simulink model "FDI_FTC_MKGMPH017"  (R2026a)
settings: Solver=ode4  StopTime=20  FixedStep=sim_dt
PreLoadFcn:
  | %% Quadrotor model parameters
  | % Initialize all model, fault detection, wind and noise settings.
  | 
  | m   = (75 + 45.7)/1000;  % kg
  | l   = 54.33e-3;  % m
  | Jxx = 54737.66e-9;  % kg m^2
  | Jyy = 53435.96e-9;  % kg m^2
  | Jzz = 98934.3e-9;  % kg m^2
  | g   = 9.81;  % m/s^2
  | 
  | %% Motor
  | 
  | kf  = 5e-8;  % N/(rad/s)^2
  | kt  = 0.025*kf;  % N m/(rad/s)^2
  | tau = 0.02;  % s
  | w_max = 2.5*sqrt(m*g/(4*kf));  % rad/s
  | 
  | %% Controller Gains
  | % Attitude controller gains
  | Kp_r = 60*Jxx;   Kd_r = 12*Jxx;  % roll
  | Kp_p = 60*Jyy;   Kd_p = 12*Jyy;  % pitch
  | Kp_y = 3*Jzz;    Kd_y = 2.5*Jzz;  % yaw
  | % Position controller gains
  | Kp_pos  = 1.2;  % [1/s^2]
  | Kd_pos  = 1.8;  % [1/s]
  | a_max   = 2.0;  % acceleration limit
  | att_lim = 25*pi/180;  % roll/pitch limit
  | 
  | %% Initial Conditions
  | p0  = [0; 0; 0];  % m        initial position [x; y; z]
  | v0  = [0; 0; 0];  % m/s      initial velocity
  | q0  = [1; 0; 0; 0];  % initial quaternion
  | om0 = [0; 0; 0];  % rad/s    initial body rates [p; q; r]
  | 
  | %% Test Scenario
  | sim_stop_time = 12;  % s
  | sim_dt        = 0.001;  % s
  | 
  | % Reference step times and values
  | x_step_time   = 3.0;   x_step_value = 10;  % m
  | y_step_time   = 5.0;   y_step_value = 10;  % m
  | z_step_time   = 0.5;   z_step_value = 10;  % m
  | psi_step_time = 7.0;   psi_step_deg = 30;  % degrees
  | psi_step_value = deg2rad(psi_step_deg);  % rad
  | 
  | %% Summary
  | w_hover = sqrt(m*g/(4*kf));
  | fprintf('quad_params: m =  % .4f kg, l = %.4f m, hover speed = %.0f rad/s (limit %.0f rad/s)\n', ...
  |         m, l, w_hover, w_max);
  | if w_hover >= w_max
  |     warning('quad_params: hover speed is above the rotor speed limit - the quad cannot hover.');
  | end
  | 
  | L1_eul = [6; 6; 6];
  | L1_om  = [12; 12; 8];
  | L1_p   = [3; 3; 3];
  | L1_v   = [4; 4; 4];
  | % Observer 2 gains
  | L2_eul = L1_eul;
  | L2_om  = L1_om;
  | L2_p   = L1_p;
  | L2_v   = L1_v;
  | rho_alpha = 0.5;
  | % Residual threshold gains
  | Ku1 = [1; 1; 1; 1; 1];
  | Ku2 = [0.05; 0.05; 0.05; 0.05; 0.05];
  | Ku3 = [0.0004; 0.0004; 0.002; 0.002; 0.002];
  | Kl1 = Ku1;
  | Kl2 = Ku2;
  | Kl3 = Ku3;
  | T_res = 0.015;
  | % Detection thresholds
  | T_flag1     = 0.01;
  | thresh_flag1 = 0.5;
  | T_flag2     = 0.1;
  | thresh_flag2 = 0.7;
  | % Confirmation time
  | t_confirm = 0.5;
  | 
  | %% Wind
  | % Wind controls
  | if ~exist('wind_seed','var'), wind_seed = 1; end
  | wind_on      = 1;
  | wind_t_start = 10;
  | wind_t_end   = 14;
  | rng(wind_seed);
  | % Gust settings
  | wind_n      = 30;
  | wind_Om_rng = [0.1 1.5];
  | wind_alt    = 10;
  | wind_W20    = 10;
  | wind_v0     = [0; 0; 0];
  | % Wind length scales and intensity
  | wind_k    = 0.177 + 0.000823*(wind_alt*3.28084);
  | wind_Lv   = wind_alt;
  | wind_Lh   = wind_Lv/wind_k^1.2;
  | wind_sigv = 0.1*wind_W20;
  | wind_sigh = wind_sigv/wind_k^0.4;
  | % Gust frequency and amplitude
  | wind_Om  = sort(wind_Om_rng(1) + diff(wind_Om_rng)*rand(3, wind_n), 2);
  | wind_Phi = 2*pi*rand(3, wind_n);
  | wind_dOm = gradient(wind_Om);
  | wind_L   = [wind_Lh; wind_Lh; wind_Lv];
  | wind_sig = [wind_sigh; wind_sigh; wind_sigv];
  | wind_PSD = zeros(3, wind_n);
  | wind_PSD(1:2,:) = (wind_sig(1:2).^2 .* 2.*wind_L(1:2)/pi) ./ (1 + (wind_L(1:2).*wind_Om(1:2,:)).^2);
  | wind_PSD(3,:)   = (wind_sig(3)^2 * 2*wind_L(3)/pi) * (1 + 3*(wind_L(3)*wind_Om(3,:)).^2) ...
  |                   ./ (1 + (wind_L(3)*wind_Om(3,:)).^2).^2;
  | wind_A = sqrt(wind_dOm .* wind_PSD);
  | % Wind drag
  | Cd_wind = 0.5*[1.0; 1.0; 0.5];
  | 
  | %% Noise and uncertainty
  | % Noise controls
  | noise_scale   = 20;
  | proc_scale    = 1;
  | noise_ctrl_on = 1;
  | noise_seed    = 1;
  | health4_final = 0;
  | % Sensor noise
  | sig_eul = 0.005*ones(3,1);
  | sig_om  = 0.005*ones(3,1);
  | sig_p   = 0.02*ones(3,1);
  | sig_v   = 0.02*ones(3,1);
  | Ts_att  = 0.004;
  | Ts_pos  = 0.02;
  | % Process noise
  | sig_pa  = 0.10*ones(3,1);
  | sig_pw  = 0.50*ones(3,1);
  | Ts_proc = 0.005;
  | % Model uncertainty
  | m_true          = m;
  | tau_true        = tau;
  | unc_thrust_gain = 1;
  | unc_M_gain      = [1;1;1];
  | unc_omdot_gain  = [1;1;1];
  | 
  | %% Observer and FTC settings
  | obs_guard = 1;
  | ftc_latch_t = 0.01;
  | ftc_rise_win = 0;
  | ftc_rise_lo = 0.3;
  | 
  | %% Integral control settings
  | Ki_pos = 0.3;
  | xi_max = 3.3;
  | pos_zone = [1; 1; 1];
  | Ki_r = 20*Jxx;
  | Ki_p = 20*Jyy;
  | xa_max = 0.3;
  | att_zone = 0.2;
InitFcn:
  | load ftc_params_x.mat; confirm_alpha = 0.7; clip_w = ftc_clip_w;
values from neighbouring files (symbols this model uses):
  ftc_clip_w = 20    [all_parameters.m]    (also in combined_params_all.m; ftc_params.mat; ftc_params_x.mat; run_lqr_design.m = clip_w)
  K_all = S_.K_all    [all_parameters.m]    (also in combined_params_all.m; fdi_ftc_test_suite.m = zeros(3,14,4); ftc_design_delta.m = zeros(3,14,4); ftc_params.mat = [-582.443942993 432.348166886 841.012077372 147.117900209 85)
  seq_all = S_.seq_all    [all_parameters.m]    (also in combined_params_all.m; fdi_ftc_test_suite.m = zeros(14,4); ftc_design_delta.m = zeros(14,4); ftc_params.mat = [-0.00271895856304 -1.55117536674e-27 0 4.31241472788e-26 -0)
  ueq_all = S_.ueq_all    [all_parameters.m]    (also in combined_params_all.m; fdi_ftc_test_suite.m = zeros(3,4); ftc_design_delta.m = zeros(3,4); ftc_params.mat = [2597.34206069  2597.34206069  3673.19636835  2597.34206069;)
settings Model: Creator=UCT  LastModifiedBy=UCT

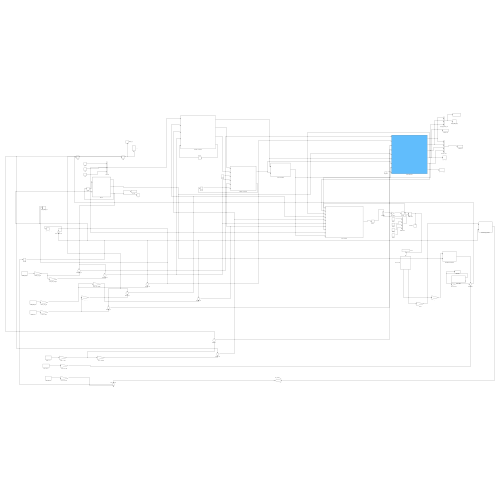
[thumbnail: Simulink's stored preview of the top-level diagram]
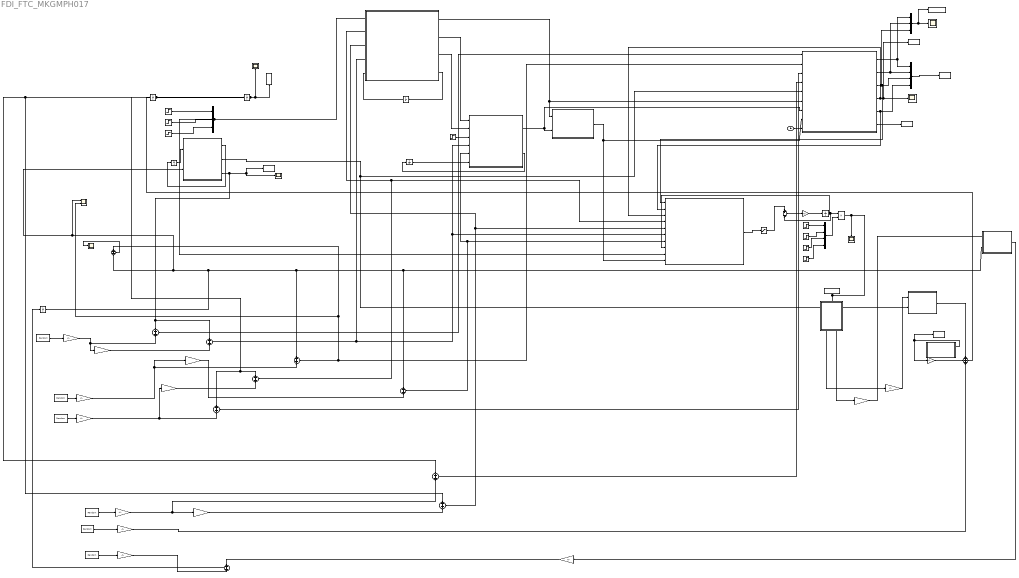
== system FDI_FTC_MKGMPH017 ==
  Att_Kin : MATLAB Function  TreatAsAtomicUnit=on
  Attitude_Controller : MATLAB Function  TreatAsAtomicUnit=on
  Control_Allocation : MATLAB Function  TreatAsAtomicUnit=on
  FD_Clock : Clock
  FD_flag_mux : Mux
  FD_flags_scope_mux : Mux  Inputs=3
  FTC_Controller : MATLAB Function  TreatAsAtomicUnit=on
  Fault_Detection : Subsystem
  Health_mux : Mux
  Health_prod : Product
  Lag_gain : Gain  Gain=1/tau_true
  Lag_int : Integrator  InitialCondition=sqrt(m*g/(4*kf))*ones(4,1)
  Lag_sum : Sum  Inputs=+-
  Position_Controller : MATLAB Function  TreatAsAtomicUnit=on
  Rotational_Dynamics : MATLAB Function  TreatAsAtomicUnit=on
  Rotor_Forces : MATLAB Function  TreatAsAtomicUnit=on
  Sat_w : Saturate  UpperLimit=w_max  LowerLimit=0
  Scope_FD_alpha : Scope
      settings: ActiveDisplayYMinimum=-0.12499999999999997  ActiveDisplayYMaximum=1.125  DataLoggingVariableName=scopedata_Scope_FD_alpha
  Scope_FD_flags : Scope
      settings: ActiveDisplayYMinimum=-0.54647490948319455  ActiveDisplayYMaximum=1.7103272831305856  DataLoggingVariableName=scopedata_Scope_FD_flags
  Scope_eul : Scope
      settings: ActiveDisplayYMinimum=-4.7929691132816243  ActiveDisplayYMaximum=4.7594431043530188  DataLoggingVariableName=scopedata_Scope_eul
  Scope_noise_only : Scope
      settings: ActiveDisplayYMinimum=-1  ActiveDisplayYMaximum=1  DataLoggingVariableName=scopedata_Scope_noise_only
  Scope_noisy_om : Scope  NumInputPorts=2
      settings: ActiveDisplayYMinimum=-1  ActiveDisplayYMaximum=1  DataLoggingVariableName=scopedata_Scope_noisy_om
  Scope_p : Scope
      settings: ActiveDisplayYMinimum=-20  ActiveDisplayYMaximum=15  DataLoggingVariableName=scopedata_Scope_p
  Scope_w : Scope
      settings: ActiveDisplayYMinimum=-1805.286321846575  ActiveDisplayYMaximum=8059.113926603749  DataLoggingVariableName=scopedata_Scope_w
  To Workspace : ToWorkspace  VariableName=flags  SaveFormat=Timeseries  SampleTime=-1
  Translational_Dynamics : MATLAB Function  TreatAsAtomicUnit=on
  Wind_Model : Subsystem
  Wind_Sum : Sum  Inputs=+++
  Wind_to_accel : Gain  Gain=1/m_true
  att_int : Integrator  InitialCondition=zeros(3,1)
  eul_log : ToWorkspace  VariableName=eul_log  SaveFormat=Timeseries  SampleTime=-1
  fd_alpha_log : ToWorkspace  VariableName=fd_alpha  SaveFormat=Timeseries  SampleTime=-1
  fd_flags_log : ToWorkspace  VariableName=fd_flags  SaveFormat=Timeseries  SampleTime=-1
  fd_residual_log : ToWorkspace  VariableName=fd_residual  SaveFormat=Timeseries  SampleTime=-1
  health_1 : Step  Time=3  InitialValue=1  SampleTime=0
  health_2 : Step  Time=15  InitialValue=1  SampleTime=0
  health_3 : Step  Time=15  InitialValue=1  SampleTime=0
  health_4 : Step  Time=15  InitialValue=1  FinalValue=0  SampleTime=0
  meas_eul_ctrl : Sum
  meas_eul_fd : Sum
  meas_om_ctrl : Sum
  meas_om_fd : Sum
  meas_p_ctrl : Sum
  meas_p_fd : Sum
  meas_v_ctrl : Sum
  meas_v_fd : Sum
  noise_check_sum : Sum  Inputs=+-
  noise_eul_ctrlgain : Gain  Gain=noise_ctrl_on
  noise_eul_gain : Gain  Gain=noise_scale*sig_eul
  noise_eul_rn : RandomNumber  Seed=noise_seed*100+10+[1 2 3]  SampleTime=Ts_att
  noise_om_ctrlgain : Gain  Gain=noise_ctrl_on
  noise_om_gain : Gain  Gain=noise_scale*sig_om
  noise_om_rn : RandomNumber  Seed=noise_seed*100+20+[1 2 3]  SampleTime=Ts_att
  noise_p_ctrlgain : Gain  Gain=noise_ctrl_on
  noise_p_gain : Gain  Gain=noise_scale*sig_p
  noise_p_rn : RandomNumber  Seed=noise_seed*100+30+[1 2 3]  SampleTime=Ts_pos
  noise_v_ctrlgain : Gain  Gain=noise_ctrl_on
  noise_v_gain : Gain  Gain=noise_scale*sig_v
  noise_v_rn : RandomNumber  Seed=noise_seed*100+40+[1 2 3]  SampleTime=Ts_pos
  om_int : Integrator  InitialCondition=om0
  p_int : Integrator  InitialCondition=p0
  p_log : ToWorkspace  VariableName=p_log  SaveFormat=Timeseries  SampleTime=-1
  p_ref_mux : Mux  Inputs=3
  pos_int : Integrator  InitialCondition=zeros(3,1)
  proc_acc_gain : Gain  Gain=proc_scale*sig_pa
  proc_acc_rn : RandomNumber  Seed=noise_seed*100+71+[1 2 3]  SampleTime=Ts_proc
  proc_om_gain : Gain  Gain=proc_scale*sig_pw
  proc_om_rn : RandomNumber  Seed=noise_seed*100+81+[1 2 3]  SampleTime=Ts_proc
  proc_om_sum : Sum
  psi_ref : Step  Time=psi_step_time  FinalValue=psi_step_value  SampleTime=0
  q_int : Integrator  InitialCondition=q0
  unc_M : Gain  Gain=unc_M_gain
  unc_omdot : Gain  Gain=unc_omdot_gain
  unc_thrust : Gain  Gain=unc_thrust_gain
  v_int : Integrator  InitialCondition=v0
  w_log : ToWorkspace  VariableName=w_log  SaveFormat=Timeseries  SampleTime=-1
  wind_log : ToWorkspace  VariableName=wind_log  SaveFormat=Timeseries  SampleTime=-1
  x_ref : Step  Time=9  FinalValue=3  SampleTime=0
  y_ref : Step  Time=6  FinalValue=-5  SampleTime=0
  z_ref : Step  Time=0.5  FinalValue=5  SampleTime=0
  wires:
  FD_flag_mux/1 -> fd_flags_log/1
  q_int/1 -> Att_Kin/1(q)
  v_int/1 -> meas_v_ctrl/1, meas_v_fd/1, p_int/1
  z_ref/1 -> p_ref_mux/3
  p_ref_mux/1 -> Position_Controller/1(p_ref), FTC_Controller/9(p_ref)
  y_ref/1 -> p_ref_mux/2
  x_ref/1 -> p_ref_mux/1
  om_int/1 -> Rotational_Dynamics/2(om), meas_om_ctrl/1, meas_om_fd/1, Att_Kin/2(om), Scope_noisy_om/1, noise_check_sum/2
  health_3/1 -> Health_mux/3
  p_int/1 -> meas_p_ctrl/1, meas_p_fd/1, p_log/1, Scope_p/1
  Att_Kin/1(q_dot) -> q_int/1
  Att_Kin/2(R) -> Fault_Detection/5(R_meas), Translational_Dynamics/2(R)
  Att_Kin/3(eul) -> meas_eul_ctrl/1, meas_eul_fd/1, eul_log/1, Scope_eul/1
  Fault_Detection/2(Flag2) -> FD_flags_scope_mux/2, FD_flag_mux/2
  Position_Controller/1(fc_des) -> Control_Allocation/1(fc_des), Fault_Detection/6(fc_nom)
  Position_Controller/2(phi_cmd) -> Attitude_Controller/1(phi_cmd)
  Position_Controller/3(theta_cmd) -> Attitude_Controller/2(theta_cmd)
  psi_ref/1 -> Attitude_Controller/3(psi_ref)
  Sat_w/1 -> Lag_sum/1
  Attitude_Controller/1(M) -> Control_Allocation/2(M), Fault_Detection/7(M_nom)
  Control_Allocation/1(w_des) -> Fault_Detection/8(w_des), FTC_Controller/10(w_nom)
  FD_Clock/1 -> Fault_Detection/9(t)
  Fault_Detection/1(Flag1) -> FD_flags_scope_mux/1, FD_flag_mux/1
  Lag_int/1 -> Lag_sum/2, Health_prod/1, FTC_Controller/8(w_act)
  Fault_Detection/3(Fault_True) -> FTC_Controller/1(Fault_True), FD_flag_mux/3, FD_flags_scope_mux/3
  Fault_Detection/4(alpha_hat) -> Scope_FD_alpha/1, fd_alpha_log/1, FTC_Controller/3(alpha_hat)
  Fault_Detection/5(faulty_rotor) -> FD_flag_mux/4, FTC_Controller/2(faulty_rotor)
  Fault_Detection/6(residual) -> fd_residual_log/1
  FD_flags_scope_mux/1 -> To Workspace/1, Scope_FD_flags/1
  Lag_sum/1 -> Lag_gain/1
  Lag_gain/1 -> Lag_int/1
  health_1/1 -> Health_mux/1
  health_2/1 -> Health_mux/2
  health_4/1 -> Health_mux/4
  Health_prod/1 -> Rotor_Forces/1(w), w_log/1, Scope_w/1
  Health_mux/1 -> Health_prod/2
  FTC_Controller/1(w_des) -> Sat_w/1
  Translational_Dynamics/1(p_ddot) -> Wind_Sum/1
  Wind_Model/1(F_wind) -> Wind_to_accel/1, wind_log/1
  Wind_to_accel/1 -> Wind_Sum/2
  Wind_Sum/1 -> v_int/1
  noise_eul_rn/1 -> noise_eul_gain/1
  noise_eul_gain/1 -> meas_eul_fd/2, noise_eul_ctrlgain/1
  noise_eul_ctrlgain/1 -> meas_eul_ctrl/2
  meas_eul_fd/1 -> Fault_Detection/1(eul_meas)
  meas_eul_ctrl/1 -> Attitude_Controller/4(eul), FTC_Controller/6(eul), Position_Controller/4(eul)
  noise_om_rn/1 -> noise_om_gain/1
  noise_om_gain/1 -> noise_om_ctrlgain/1, meas_om_fd/2
  noise_om_ctrlgain/1 -> meas_om_ctrl/2
  meas_om_fd/1 -> noise_check_sum/1, Scope_noisy_om/2, Fault_Detection/2(om_meas)
  meas_om_ctrl/1 -> Attitude_Controller/5(om), FTC_Controller/7(om)
  noise_p_rn/1 -> noise_p_gain/1
  noise_p_gain/1 -> noise_p_ctrlgain/1, meas_p_fd/2
  noise_p_ctrlgain/1 -> meas_p_ctrl/2
  meas_p_fd/1 -> Fault_Detection/3(p_meas)
  meas_p_ctrl/1 -> Position_Controller/2(p), FTC_Controller/4(p)
  noise_v_rn/1 -> noise_v_gain/1
  noise_v_gain/1 -> meas_v_fd/2, noise_v_ctrlgain/1
  noise_v_ctrlgain/1 -> meas_v_ctrl/2
  meas_v_fd/1 -> Fault_Detection/4(v_meas)
  meas_v_ctrl/1 -> Position_Controller/3(v), FTC_Controller/5(v)
  proc_acc_rn/1 -> proc_acc_gain/1
  proc_acc_gain/1 -> Wind_Sum/3
  Rotational_Dynamics/1(om_dot) -> unc_omdot/1
  unc_omdot/1 -> proc_om_sum/1
  proc_om_gain/1 -> proc_om_sum/2
  proc_om_rn/1 -> proc_om_gain/1
  proc_om_sum/1 -> om_int/1
  Rotor_Forces/1(f) -> unc_thrust/1
  unc_thrust/1 -> Translational_Dynamics/1(f)
  Rotor_Forces/2(M) -> unc_M/1
  unc_M/1 -> Rotational_Dynamics/1(M)
  noise_check_sum/1 -> Scope_noise_only/1
  Position_Controller/4(dxi) -> pos_int/1
  pos_int/1 -> Position_Controller/5(xi)
  Attitude_Controller/2(dxa) -> att_int/1
  att_int/1 -> Attitude_Controller/6(xa)

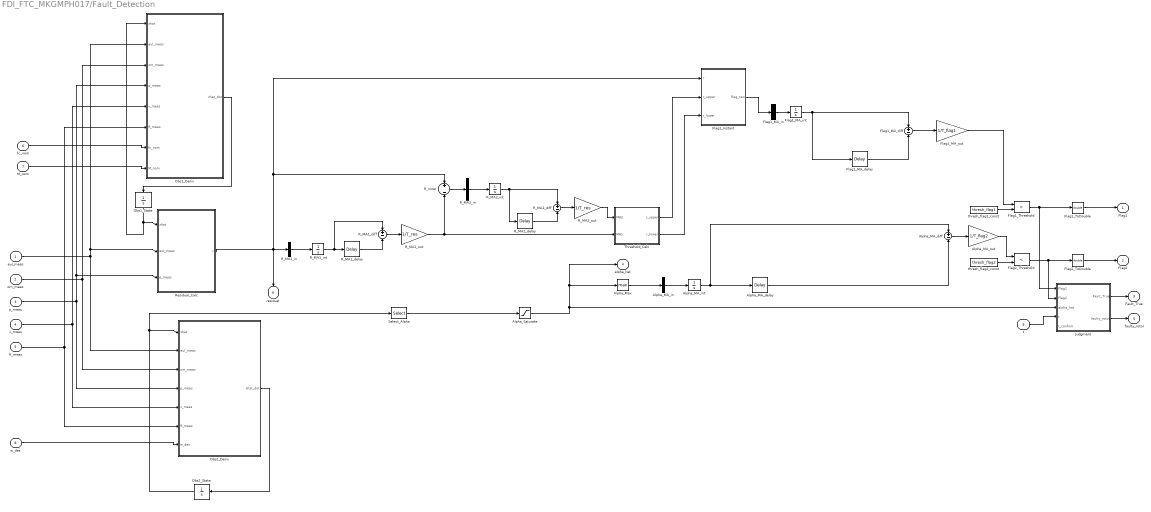
== system FDI_FTC_MKGMPH017/Fault_Detection ==
  eul_meas : Inport
  om_meas : Inport  Port=2
  p_meas : Inport  Port=3
  v_meas : Inport  Port=4
  R_meas : Inport  Port=5
  fc_nom : Inport  Port=6
  M_nom : Inport  Port=7
  w_des : Inport  Port=8
  t : Inport  Port=9
  Alpha_MA_delay : TransportDelay  DelayTime=T_flag2
  Alpha_MA_diff : Sum  Inputs=+-
  Alpha_MA_in : Mux  Inputs=1
  Alpha_MA_int : Integrator
  Alpha_MA_out : Gain  Gain=1/T_flag2
  Alpha_Max : MinMax  Function=max
  Alpha_Saturate : Saturate  UpperLimit=1  LowerLimit=0
  Flag1_Instant : MATLAB Function  TreatAsAtomicUnit=on
  Flag1_MA_delay : TransportDelay  DelayTime=T_flag1
  Flag1_MA_diff : Sum  Inputs=+-
  Flag1_MA_in : Mux  Inputs=1
  Flag1_MA_int : Integrator
  Flag1_MA_out : Gain  Gain=1/T_flag1
  Flag1_Threshold : RelationalOperator  Operator=>  OutDataTypeStr=boolean  RndMeth=Simplest  InputSameDT=off
  Flag1_ToDouble : DataTypeConversion  OutDataTypeStr=double  SaturateOnIntegerOverflow=off  RndMeth=Floor
  Flag2_Threshold : RelationalOperator  Operator=<  OutDataTypeStr=boolean  RndMeth=Simplest  InputSameDT=off
  Flag2_ToDouble : DataTypeConversion  OutDataTypeStr=double  SaturateOnIntegerOverflow=off  RndMeth=Floor
  Judgment : MATLAB Function  TreatAsAtomicUnit=on
  Obs1_Deriv : MATLAB Function  TreatAsAtomicUnit=on
  Obs1_State : Integrator  InitialCondition=zeros(12,1)
  Obs2_Deriv : MATLAB Function  TreatAsAtomicUnit=on
  Obs2_State : Integrator  InitialCondition=zeros(16,1)
  R_MA1_delay : TransportDelay  DelayTime=T_res  InitialOutput=zeros(5,1)
  R_MA1_diff : Sum  Inputs=+-
  R_MA1_in : Mux  Inputs=1
  R_MA1_int : Integrator  InitialCondition=zeros(5,1)
  R_MA1_out : Gain  Gain=1/T_res
  R_MA2_delay : TransportDelay  DelayTime=T_res  InitialOutput=zeros(5,1)
  R_MA2_diff : Sum  Inputs=+-
  R_MA2_in : Mux  Inputs=1
  R_MA2_int : Integrator  InitialCondition=zeros(5,1)
  R_MA2_out : Gain  Gain=1/T_res
  R_inner : Sum  Inputs=+-
  Residual_Calc : MATLAB Function  TreatAsAtomicUnit=on
  Select_Alpha : Selector  InputPortWidth=16  IndexOptions=Index vector (dialog)  Indices=[13 14 15 16]  OutputSizes=1
  Threshold_Calc : MATLAB Function  TreatAsAtomicUnit=on
  thresh_flag1_const : Constant  Value=thresh_flag1
  thresh_flag2_const : Constant  Value=thresh_flag2
  Flag1 : Outport
  Flag2 : Outport  Port=2
  Fault_True : Outport  Port=3
  alpha_hat : Outport  Port=4
  faulty_rotor : Outport  Port=5
  residual : Outport  Port=6
  wires:
  Flag2_ToDouble/1 -> Flag2/1
  Obs2_State/1 -> Obs2_Deriv/1(xhat), Select_Alpha/1
  R_meas/1 -> Obs1_Deriv/6(R_meas), Obs2_Deriv/6(R_meas)
  Alpha_Saturate/1 -> alpha_hat/1, Alpha_Max/1, Judgment/3(alpha_hat)
  R_MA2_int/1 -> R_MA2_delay/1, R_MA2_diff/1
  v_meas/1 -> Obs2_Deriv/5(v_meas), Obs1_Deriv/5(v_meas)
  Residual_Calc/1(r) -> Flag1_Instant/1(r), R_inner/1, residual/1, R_MA1_in/1
  p_meas/1 -> Obs1_Deriv/4(p_meas), Residual_Calc/3(p_meas), Obs2_Deriv/4(p_meas)
  om_meas/1 -> Obs2_Deriv/3(om_meas), Obs1_Deriv/3(om_meas)
  M_nom/1 -> Obs1_Deriv/8(M_nom)
  fc_nom/1 -> Obs1_Deriv/7(fc_nom)
  Flag1_MA_delay/1 -> Flag1_MA_diff/2
  Obs1_State/1 -> Obs1_Deriv/1(xhat), Residual_Calc/1(xhat)
  thresh_flag2_const/1 -> Flag2_Threshold/2
  eul_meas/1 -> Residual_Calc/2(eul_meas), Obs1_Deriv/2(eul_meas), Obs2_Deriv/2(eul_meas)
  Judgment/1(Fault_True) -> Fault_True/1
  w_des/1 -> Obs2_Deriv/7(w_des)
  Obs1_Deriv/1(xhat_dot) -> Obs1_State/1
  Obs2_Deriv/1(xhat_dot) -> Obs2_State/1
  R_MA1_in/1 -> R_MA1_int/1
  R_MA1_int/1 -> R_MA1_diff/1, R_MA1_delay/1
  Select_Alpha/1 -> Alpha_Saturate/1
  Flag2_Threshold/1 -> Flag2_ToDouble/1, Judgment/2(Flag2)
  R_MA1_delay/1 -> R_MA1_diff/2
  R_MA1_diff/1 -> R_MA1_out/1
  Alpha_MA_delay/1 -> Alpha_MA_diff/2
  Alpha_Max/1 -> Alpha_MA_in/1
  R_MA1_out/1 -> Threshold_Calc/2(MA1), R_inner/2
  Flag1_MA_in/1 -> Flag1_MA_int/1
  R_inner/1 -> R_MA2_in/1
  R_MA2_in/1 -> R_MA2_int/1
  Alpha_MA_in/1 -> Alpha_MA_int/1
  R_MA2_delay/1 -> R_MA2_diff/2
  R_MA2_diff/1 -> R_MA2_out/1
  Threshold_Calc/1(r_upper) -> Flag1_Instant/2(r_upper)
  Threshold_Calc/2(r_lower) -> Flag1_Instant/3(r_lower)
  Flag1_ToDouble/1 -> Flag1/1
  Flag1_Instant/1(flag_raw) -> Flag1_MA_in/1
  Flag1_Threshold/1 -> Flag1_ToDouble/1, Judgment/1(Flag1)
  Flag1_MA_int/1 -> Flag1_MA_delay/1, Flag1_MA_diff/1
  Alpha_MA_int/1 -> Alpha_MA_diff/1, Alpha_MA_delay/1
  Flag1_MA_diff/1 -> Flag1_MA_out/1
  Judgment/2(faulty_rotor) -> faulty_rotor/1
  Alpha_MA_diff/1 -> Alpha_MA_out/1
  Flag1_MA_out/1 -> Flag1_Threshold/1
  thresh_flag1_const/1 -> Flag1_Threshold/2
  t/1 -> Judgment/4(t)
  Alpha_MA_out/1 -> Flag2_Threshold/1
  R_MA2_out/1 -> Threshold_Calc/1(MA2)

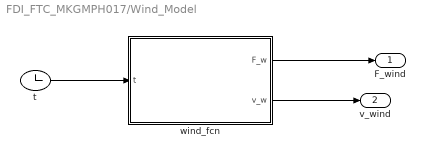
== system FDI_FTC_MKGMPH017/Wind_Model ==
  t : Clock
  wind_fcn : MATLAB Function  TreatAsAtomicUnit=on
  F_wind : Outport
  v_wind : Outport  Port=2
  wires:
  t/1 -> wind_fcn/1(t)
  wind_fcn/1(F_w) -> F_wind/1
  wind_fcn/2(v_w) -> v_wind/1

== matlab function FDI_FTC_MKGMPH017/Att_Kin ==
  data: q input; q_dot output; om input; R output; eul output
function [q_dot, R, eul] = att_kin(q, om)
qv = q(:); o = om(:);
qn = qv/norm(qv); %normalising  
qa = qn(1); q1 = qn(2); q2 = qn(3); q3 = qn(4);
p = o(1); qq = o(2); r = o(3);

%quaternion multiplication 
q_dot = 0.5*[-q1*p - q2*qq - q3*r; ...
              qa*p + q2*r - q3*qq; ...
              qa*qq - q1*r + q3*p; ...
              qa*r + q1*qq - q2*p];
%quaternion to rotational matrix 
R = [1-2*(q2^2+q3^2), 2*(q1*q2-qa*q3),   2*(q1*q3+qa*q2); ...
     2*(q1*q2+qa*q3), 1-2*(q1^2+q3^2),   2*(q2*q3-qa*q1); ...
     2*(q1*q3-qa*q2), 2*(q2*q3+qa*q1),   1-2*(q1^2+q2^2)];

%quaternion to euler 
phi   = atan2(2*(qa*q1+q2*q3), 1-2*(q1^2+q2^2));
theta = asin(max(-1, min(1, 2*(qa*q2-q3*q1))));
psi   = atan2(2*(qa*q3+q1*q2), 1-2*(q2^2+q3^2));
eul = [phi; theta; psi];
end

== matlab function FDI_FTC_MKGMPH017/Translational_Dynamics ==
  data: f input; p_ddot output; R input; m parameter; g parameter
function p_ddot = trans_dyn(f, R, m, g)
% m*p_ddot = WR_B*[0;0;f] + [0;0;-m*g]
p_ddot = (R*[0; 0; f] + [0; 0; -m*g])/m;
end

== matlab function FDI_FTC_MKGMPH017/Fault_Detection/Obs1_Deriv ==
  data: xhat input; xhat_dot output; eul_meas input; om_meas input; p_meas input; v_meas input; R_meas input; fc_nom input; M_nom input; Jxx parameter; Jyy parameter; Jzz parameter; m parameter; g parameter; L1_eul parameter; L1_om parameter; L1_p parameter; L1_v parameter; obs_guard parameter
function xhat_dot = obs1_deriv(xhat, eul_meas, om_meas, p_meas, v_meas, R_meas, fc_nom, M_nom, Jxx, Jyy, Jzz, m, g, L1_eul, L1_om, L1_p, L1_v, obs_guard)


eul_hat = xhat(1:3); om_hat = xhat(4:6); p_hat = xhat(7:9); v_hat = xhat(10:12);
if obs_guard > 0.5
    om_hat = max(min(om_hat, 300), -300);
end
phi = eul_hat(1); theta = eul_hat(2);
cth = cos(theta); cth = sign(cth + (cth==0))*max(abs(cth), 1e-3);
tth = tan(theta);  if obs_guard > 0.5, tth = sin(theta)/cth; end %avoids dividing by zero when pitch is at 90

H = [1, sin(phi)*tth, cos(phi)*tth; ...
     0, cos(phi),           -sin(phi); ...
     0, sin(phi)/cth,        cos(phi)/cth];

Jv = [Jxx; Jyy; Jzz];
dE = eul_meas - eul_hat;  if obs_guard > 0.5, dE = atan2(sin(dE), cos(dE)); end

%EQ3 additional terms are neglected as many papers also neglect the effects of the propellers
om_dot_nom = (M_nom - cross(om_hat, Jv.*om_hat)) ./ Jv; 

%state estimation error 
eul_hat_dot = H*om_hat  + L1_eul.*dE; 
om_hat_dot  = om_dot_nom + L1_om.*(om_meas  - om_hat);
p_hat_dot   = v_hat      + L1_p.*(p_meas    - p_hat);
v_hat_dot   = (R_meas*[0;0;fc_nom/m] - [0;0;g]) + L1_v.*(v_meas - v_hat);


xhat_dot = [eul_hat_dot; om_hat_dot; p_hat_dot; v_hat_dot]; % state vector 
if obs_guard > 0.5
    xhat_dot(~isfinite(xhat_dot)) = 0;
    xhat_dot = max(min(xhat_dot, 1e6), -1e6);
end
end

== matlab function FDI_FTC_MKGMPH017/Fault_Detection/Residual_Calc ==
  data: xhat input; r output; eul_meas input; p_meas input; obs_guard parameter
function r = residual_calc(xhat, eul_meas, p_meas, obs_guard)
eul_hat = xhat(1:3); p_hat = xhat(7:9);
r = [eul_meas(1) - eul_hat(1); ... %roll
     eul_meas(2) - eul_hat(2); ... %pitch 
     p_meas      - p_hat];
if obs_guard > 0.5, r(1:2) = atan2(sin(r(1:2)), cos(r(1:2))); end         % x, y ,z 
end

% The residual for the yaw is not calculated

== matlab function FDI_FTC_MKGMPH017/Fault_Detection/Threshold_Calc ==
  data: MA2 input; MA1 input; r_upper output; r_lower output; Ku1 parameter; Ku2 parameter; Ku3 parameter; Kl1 parameter; Kl2 parameter; Kl3 parameter
function [r_upper, r_lower] = threshold_calc(MA2, MA1, Ku1, Ku2, Ku3, Kl1, Kl2, Kl3)
% Paper Eq. 38-39 adaptive residue boundary, per-state gains from Table 2
r_upper = Ku1.*MA1 + Ku2.*MA2 + Ku3;
r_lower = Kl1.*MA1 + Kl2.*MA2 - Kl3;
end

== matlab function FDI_FTC_MKGMPH017/Fault_Detection/Flag1_Instant ==
  data: r input; flag_raw output; r_upper input; r_lower input
function flag_raw= flag1_instant(r, r_upper, r_lower)
exceed = any(r > r_upper) || any(r < r_lower);
flag_raw = double(~exceed);   %% 1 = normal, 0 = exceeds bound
end

== matlab function FDI_FTC_MKGMPH017/Fault_Detection/Obs2_Deriv ==
  data: xhat input; xhat_dot output; eul_meas input; om_meas input; p_meas input; v_meas input; R_meas input; w_des input; Jxx parameter; Jyy parameter; Jzz parameter; m parameter; g parameter; kf parameter; kt parameter; l parameter; L2_eul parameter; L2_om parameter; L2_p parameter; L2_v parameter; rho_alpha parameter; obs_guard parameter
function xhat_dot = obs2_deriv(xhat, eul_meas, om_meas, p_meas, v_meas, R_meas, w_des, Jxx, Jyy, Jzz, m, g, kf, kt, l, L2_eul, L2_om, L2_p, L2_v, rho_alpha, obs_guard)

%the start is the same as observer 1
eul_hat = xhat(1:3); om_hat = xhat(4:6); p_hat = xhat(7:9); v_hat = xhat(10:12);
a_hat = xhat(13:16);
if obs_guard > 0.5
    om_hat = max(min(om_hat, 300), -300);
    a_hat = max(min(a_hat, 1), 0);
end
phi = eul_hat(1); theta = eul_hat(2);
cth = cos(theta); cth = sign(cth + (cth==0))*max(abs(cth), 1e-3);
tth = tan(theta);  if obs_guard > 0.5, tth = sin(theta)/cth; end
H = [1, sin(phi)*tth, cos(phi)*tth; ...
     0, cos(phi),           -sin(phi); ...
     0, sin(phi)/cth,        cos(phi)/cth];
Jv = [Jxx; Jyy; Jzz];
dE = eul_meas - eul_hat;  if obs_guard > 0.5, dE = atan2(sin(dE), cos(dE)); end


f_nom = kf*w_des.^2;                 %% 4x1 commanded per-rotor thrust
f1 = f_nom(1); f2 = f_nom(2); f3 = f_nom(3); f4 = f_nom(4);

%predicted actual net force/moment given current fault estimate
f_pred  = sum(f_nom) - sum(a_hat.*f_nom);
Mx_pred = (l/sqrt(2))*((-f1 - f2 + f3 + f4) - (-a_hat(1)*f1 - a_hat(2)*f2 + a_hat(3)*f3 + a_hat(4)*f4));
My_pred = (l/sqrt(2))*((-f1 + f2 + f3 - f4) - (-a_hat(1)*f1 + a_hat(2)*f2 + a_hat(3)*f3 - a_hat(4)*f4));
Mz_pred = (kt/kf)*((f1-f2+f3-f4) - (a_hat(1)*f1 - a_hat(2)*f2 + a_hat(3)*f3 - a_hat(4)*f4));
M_pred  = [Mx_pred; My_pred; Mz_pred];


%state estimation error
om_dot_pred = (M_pred - cross(om_hat, Jv.*om_hat)) ./ Jv;
eul_hat_dot = H*om_hat  + L2_eul.*dE;
om_hat_dot  = om_dot_pred + L2_om.*(om_meas - om_hat);
p_hat_dot   = v_hat      + L2_p.*(p_meas   - p_hat);
v_hat_dot   = (R_meas*[0;0;f_pred/m] - [0;0;g]) + L2_v.*(v_meas - v_hat);

% gradient update for alpha_hat (MIT-rule style, projected to [0,1])
e_om = om_meas - om_hat;
e_v  = v_meas  - v_hat;
S_Mx = (l/sqrt(2))*[f1, f2, -f3, -f4];
S_My = (l/sqrt(2))*[f1, -f2, -f3, f4];
S_Mz = (kt/kf)*[-f1, f2, -f3, f4];
S_f  = -f_nom(:)';
a_dot = zeros(4,1);
for i = 1:4
    dOmdA = [S_Mx(i); S_My(i); S_Mz(i)] ./ Jv;
    dVdA  = R_meas*[0; 0; S_f(i)/m];
    a_dot(i) = rho_alpha*(dOmdA'*e_om + dVdA'*e_v); %Lyapunov equation
    if (a_hat(i) >= 1 && a_dot(i) > 0) || (a_hat(i) <= 0 && a_dot(i) < 0)
        a_dot(i) = 0;   % simple projection to keep alpha_hat in [0,1]
    end
end

xhat_dot = [eul_hat_dot; om_hat_dot; p_hat_dot; v_hat_dot; a_dot];
if obs_guard > 0.5
    xhat_dot(~isfinite(xhat_dot)) = 0;
    xhat_dot = max(min(xhat_dot, 1e6), -1e6);
end
end

== matlab function FDI_FTC_MKGMPH017/Fault_Detection/Judgment ==
  settings: updateMethod=DISCRETE
  data: Flag1 input; Fault_True output; Flag2 input; alpha_hat input; t input; faulty_rotor output; t_confirm input
function [Fault_True, faulty_rotor] = judgment(Flag1, Flag2, alpha_hat, t, t_confirm)


persistent FaultTrue tOkStart
if isempty(FaultTrue)
    FaultTrue = false;
    tOkStart = -1;
end
bothOk = (Flag1 >= 1) && (Flag2 >= 1);
if ~FaultTrue
    if (Flag1 < 1) || (Flag2 < 1)
        FaultTrue = true;
        tOkStart = -1;
    end
else
    if bothOk
        if tOkStart < 0
            tOkStart = t;
        elseif (t - tOkStart) >= t_confirm
            FaultTrue = false;
            tOkStart = -1;
        end
    else
        tOkStart = -1;
    end
end
if FaultTrue
    [~, faulty_rotor] = max(alpha_hat);
else
    faulty_rotor = 0;
end
Fault_True = double(FaultTrue);
end

== matlab function FDI_FTC_MKGMPH017/FTC_Controller ==
  settings: updateMethod=DISCRETE
  data: Fault_True input; w_des output; faulty_rotor input; alpha_hat input; p input; v input; eul input; om input; w_act input; p_ref input; w_nom input; K_all parameter; seq_all parameter; ueq_all parameter; clip_w parameter; confirm_alpha parameter; ftc_latch_t parameter; ftc_rise_win parameter; ftc_rise_lo parameter; sim_dt parameter
function w_des = ftc_controller(Fault_True, faulty_rotor, alpha_hat, p, v, eul, om, w_act, p_ref, w_nom, ...
                                K_all, seq_all, ueq_all, clip_w, confirm_alpha, ftc_latch_t, ftc_rise_win, ftc_rise_lo, sim_dt)
% MATLAB Function block. Passes the normal allocation w_nom through until a rotor failure is
% CONFIRMED, then latches the failed rotor and runs the spinning-hover LQR on the other three.
%   p,v,p_ref : 3x1 world position / velocity / position reference
%   eul       : [phi;theta;psi] ;  om : body rates ;  w_act : 4x1 actual rotor speeds (lag output)
%   w_nom     : 4x1 output of Control_Allocation ;  K_all/seq_all/ueq_all from ftc_design.m
persistent k_lat n_ok k_cand abuf
if isempty(k_lat), k_lat = 0; n_ok = 0; k_cand = 0; abuf = zeros(4,256); end
abuf = [abuf(:,2:end), alpha_hat(:)];            % last 256 samples of the thrust-loss estimates
if k_lat == 0
    kk = max(1, round(faulty_rotor));
    ok = Fault_True > 0.5 && faulty_rotor >= 1 && alpha_hat(kk) > confirm_alpha;
    if ok && ftc_rise_win > 0          % the estimate must have risen from a low value recently
        nw = min(256, max(1, round(ftc_rise_win/sim_dt)));
        ok = min(abuf(kk, end-nw+1:end)) < ftc_rise_lo;
    end
    if ok && kk == k_cand, n_ok = n_ok + 1; elseif ok, n_ok = 1; k_cand = kk; else, n_ok = 0; k_cand = 0; end
    if ok && n_ok*sim_dt >= ftc_latch_t - 1e-12
        k_lat = kk;                    % latch: a dead rotor does not come back
    end
end
if k_lat == 0
    w_des = w_nom;  return;
end
live = 1:4;  live(k_lat) = [];
c = cos(eul(3)); s = sin(eul(3));  Rz = [c s 0; -s c 0; 0 0 1];   % world -> yaw-rotating frame
sv  = [Rz*(p(:)-p_ref(:)); Rz*v(:); eul(1); eul(2); om(:); w_act(live)];
err = sv - seq_all(:,k_lat);
err(9:11) = min(max(err(9:11), -clip_w), clip_w);      % rate-error clip -> smooth spin-up
err(1:3) = min(max(err(1:3), -2), 2);   % limit position error to 2 m
wc  = ueq_all(:,k_lat) - K_all(:,:,k_lat)*err;
w_des = zeros(4,1);  w_des(live) = wc;                 % failed rotor commanded to 0
end

== matlab function FDI_FTC_MKGMPH017/Wind_Model/wind_fcn ==
  data: t input; F_w output; v_w output; wind_A parameter; wind_Om parameter; wind_Phi parameter; wind_v0 parameter; Cd_wind parameter; wind_on parameter; wind_t_start parameter; wind_t_end parameter
function [F_w, v_w] = wind_fcn(t, wind_A, wind_Om, wind_Phi, wind_v0, Cd_wind, wind_on, wind_t_start, wind_t_end)
v_w = wind_v0 + sum(wind_A .* sin(wind_Om*t + wind_Phi), 2);
F_w = wind_on * (t >= wind_t_start && t <= wind_t_end) * (Cd_wind .* v_w);
end

== matlab function FDI_FTC_MKGMPH017/Attitude_Controller ==
  data: phi_cmd input; M output; theta_cmd input; psi_ref input; eul input; om input; Kp_r parameter; Kd_r parameter; Kp_p parameter; Kd_p parameter; Kp_y parameter; Kd_y parameter; xa input; dxa output; Ki_r parameter; Ki_p parameter; xa_max parameter; att_zone parameter
function [M, dxa] = attitude_controller(phi_cmd, theta_cmd, psi_ref, eul, om, Kp_r, Kd_r, Kp_p, Kd_p, Kp_y, Kd_y, xa, Ki_r, Ki_p, xa_max, att_zone)
e = eul(:); o = om(:);
e_psi = atan2(sin(psi_ref - e(3)), cos(psi_ref - e(3)));   % wrapped yaw error
Mx = Kp_r*(phi_cmd   - e(1)) - Kd_r*o(1) + Ki_r*xa(1);
My = Kp_p*(theta_cmd - e(2)) - Kd_p*o(2) + Ki_p*xa(2);
e_a = [phi_cmd - e(1); theta_cmd - e(2); 0];
dxa = e_a;                                              % integral of the roll / pitch error (yaw: none)
for i = 1:2
    if abs(e_a(i)) > att_zone || (abs(xa(i)) >= xa_max && xa(i)*e_a(i) > 0)
        dxa(i) = 0;                                     % anti-windup
    end
end
Mz = Kp_y*e_psi           - Kd_y*o(3);
M = [Mx; My; Mz];
end

% checks the command pitch, roll and yaw angles respective to where they
% have to be and then outputs the torque required to correct the error is
% there is

== matlab function FDI_FTC_MKGMPH017/Position_Controller ==
  data: p_ref input; fc_des output; p input; v input; eul input; phi_cmd output; theta_cmd output; Kp_pos parameter; Kd_pos parameter; a_max parameter; att_lim parameter; g parameter; m parameter; xi input; dxi output; Ki_pos parameter; xi_max parameter; pos_zone parameter
function [fc_des, phi_cmd, theta_cmd, dxi] = position_controller(p_ref, p, v, eul, Kp_pos, Kd_pos, a_max, att_lim, g, m, xi, Ki_pos, xi_max, pos_zone)

% check where the quadcopter is with respect to where it has to be and then.
% outputs the desired thrust and pitch and roll angles 

pr = p_ref(:); pp = p(:); vv = v(:); e = eul(:);
phi = e(1); theta = e(2); psi = e(3);
e_p = pr - pp;
a_raw = Kp_pos*e_p - Kd_pos*vv + Ki_pos*xi(:);          % PD + integral
a = max(min(a_raw, a_max), -a_max);
dxi = e_p;                                              % integral of the position error
for i = 1:3
    if abs(e_p(i)) > pos_zone(i) || (abs(a_raw(i)) > a_max && a_raw(i)*e_p(i) > 0) || (abs(xi(i)) >= xi_max && xi(i)*e_p(i) > 0)
        dxi(i) = 0;                                     % anti-windup
    end
end
lim = att_lim;

% rotate desired x/y acceleration into the yaw-aligned frame, small-angle map
theta_cmd = max(min((a(1)*cos(psi) + a(2)*sin(psi))/g, lim), -lim);
phi_cmd   = max(min((a(1)*sin(psi) - a(2)*cos(psi))/g, lim), -lim);

% collective thrust with tilt compensation
fc_des = m*(g + a(3))/max(cos(phi)*cos(theta), 0.5);
end

== matlab function FDI_FTC_MKGMPH017/Control_Allocation ==
  data: fc_des input; w_des output; M input; kf parameter; kt parameter; l parameter
function w_des = control_allocation(fc_des, M, kf, kt, l)
Mv = M(:);
Mx = Mv(1); My = Mv(2); Mz = Mv(3);
c = l*kf/sqrt(2);
w1sq = fc_des/(4*kf) - (Mx + My)/(4*c) + Mz/(4*kt);
w2sq = fc_des/(4*kf) - (Mx - My)/(4*c) - Mz/(4*kt);
w3sq = fc_des/(4*kf) + (Mx + My)/(4*c) + Mz/(4*kt);
w4sq = fc_des/(4*kf) + (Mx - My)/(4*c) - Mz/(4*kt);
w_des = sqrt(max([w1sq; w2sq; w3sq; w4sq], 0));
end

== matlab function FDI_FTC_MKGMPH017/Rotor_Forces ==
  data: w input; f output; M output; kf parameter; kt parameter; l parameter
function [f, M] = rotor_forces(w, kf, kt, l)
w2 = w(:).^2;
f = kf*sum(w2);
M = [(l/sqrt(2))*kf*(-w2(1) - w2(2) + w2(3) + w2(4)); ...
     (l/sqrt(2))*kf*(-w2(1) + w2(2) + w2(3) - w2(4)); ...
     kt*(w2(1) - w2(2) + w2(3) - w2(4))];
end

%It takes the four rotor speeds and returns the total thrust and the three body torques that those speeds produce.

== matlab function FDI_FTC_MKGMPH017/Rotational_Dynamics ==
  data: M input; om_dot output; om input; Jxx parameter; Jyy parameter; Jzz parameter
function om_dot = rot_dyn(M, om, Jxx, Jyy, Jzz)
% J*om_dot + om x (J*om) = M   (J diagonal)
Mv = M(:); o = om(:);
Jv = [Jxx; Jyy; Jzz];
om_dot = (Mv - cross(o, Jv.*o))./Jv;
end
